simulink model "waypoiont"  (R2026b)
settings: Solver=VariableStepAuto
undefined symbols (not defined in the file): Sim3dSensor
libraries: sim3dcameralib x1, sim3dlib x1, uavsim3dlib x1, uavalgslib x1
settings Model: Creator=Shobhit  LastModifiedBy=Shobhit

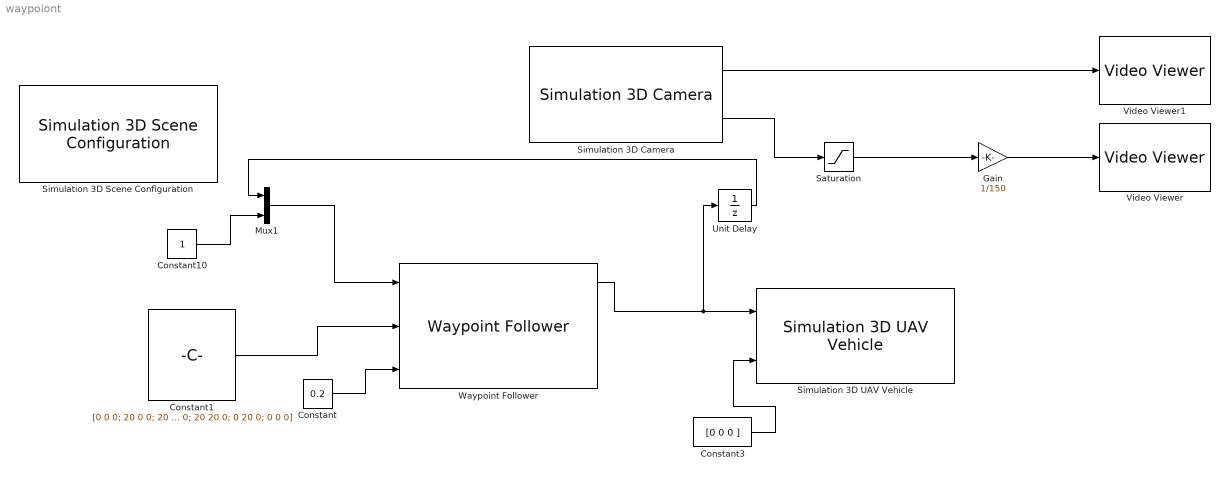
== system waypoiont ==
  Constant : Constant  Value=0.2
  Constant1 : Constant  Value=[0 0 0; 20 0 0; 20 20 0; 0 20 0; 0 0 0; 20 0 0; 20 20 0; 0 20 0; 0 0 0; 20 0 0; 20 20 0; 0 20 0; 0 0 0]
  Constant10 : Constant
  Constant3 : Constant  Value=[0 0 0 ]
  Gain : Gain  Gain=1/150
  Mux1 : Mux  Inputs=2
  Saturation : Saturate  UpperLimit=150  LowerLimit=0
  Simulation 3D Camera : sim3dcameralib/Simulation 3D Camera  Priority=1  sensorTag=Sim3dSensor�  sensorId=4  sensorName=Sim3dSensor�  vehTagList={'Custom ...';'Scene Origin';'SimulinkVehicle3'}  vehTag=SimulinkVehicle3  CoordinateSystem=Default  mountLoc=Origin  offsetFlag=off  tmountOffset=[0, 0, 0]  extTmount=off  rmountOffset=[0, 0, 0]  extRmount=off  FocalLength=[1109, 1109]  OpticalCenter=[640, 360]  ImageSize=[720, 1280]  RadialDistortion=[0, 0]  TangentialDistortion=[0, 0]  SensorSkew=0  VisualizeFieldOfView=off  FieldOfViewRange=61  DepthOutportEnabled=on  SemanticOutportEnabled=off  TransformOutportEnabled=off  SampleTime=-1  mountPoint=[0 0 0]  mountOrientation=[0 0 0]  aMode=5  ID=4
      settings: LibrarySourceBlock=sl3dlib/Simulation 3D/Sensors/Simulation 3D Camera
  Simulation 3D Scene Configuration : sim3dlib/Simulation 3D Scene Configuration  Priority=0  EnableWindow=on  ViewerType=Default Viewer  ProjectFormat=Default Scenes  SceneDesc=US city block  ProjectName=C:\Program Files\MATLAB\R2026b\toolbox\shared\sim3d_projects\automotive_project_windows\UE\WindowsNoEditor\VehicleSimulation.exe  ScenePath=/Game/Maps/USCityBlock  EnableOpenDRIVE=off  vehTagList={'Custom';'Scene Origin';'SimulinkVehicle1';'SimulinkVehicle2';'SimulinkVehicle3'}  vehTag=SimulinkVehicle3  AttachedCameraRelativeTranslation=[0 0 0]  FreeCameraDefaultInitialTranslation=[-6, 0, 2]  AttachedCameraRelativeRotation=[0, -15, 0]  FreeCameraDefaultInitialRotation=[0, -15, 0]  ViewpointName=Custom  FreeCameraInitialTranslation=[0, 0, 0]  FreeCameraInitialRotation=[0, 0, 0]  OpVisEn=off  Ts=1/60  EnableRemoteAccess=off  SimulationMode=CoSimulation  SimulateUsing=Interpreted execution  EnableAnimationRecording=off  OverrideDefaultRecording=off  AnimationRecordingFileName=sim3dAnimation.mat  AnimationRecordingInterval=[0 inf]  EnableWeather=off  SunAzimuth=90  SunAltitude=40.0  EnableGeospatialSun=off  Latitude=0  Longitude=0  Date=2023-01-01  Time=10:30:00  GeoTimeZone=-5.0  SunDaylightSaving=off  wind=1  clouds=10  EnableVolumetricClouds=off  CloudCoverage=0  CloudAltitude=6  fog=0  rain=0  RaindropsEffect=off  SnowDensity=0  EnableGeospatial=off  TilesetSource=Earth terrain  UseTrueOrigin=off  OriginHeight=200  OriginLatitude=40.744652  OriginLongitude=-73.988864  MapStyle=Aerial  AdditionalAssetIDs=[]  UseAdvancedSunSky=off  SolarTime=11  TimeZone=-5  Day=21  Month=9  Year=2022  UseDaylightSavingTime=on  DSTStartDay=10  DSTStartMonth=3  DSTEndDay=3  DSTEndMonth=11  DSTSwitchHour=2  sensorTag=MainCamera3  sensorId=3  sensorName=MainCamera3  mountLoc=Origin  offsetFlag=off  tmountOffset=[0, 0, 0]  rmountOffset=[0, 0, 0]  HorizontalResolution=1280  VerticalResolution=720  HorizontalFOV=60  mountPoint=[0 0 0]  mountOrientation=[0 0 0]  aMode=4  ID=3  GeoTrigger=Inactive  ViewNameList={'Custom'}  ViewTranslationList={'[0 0 0]'}  ViewRotationList={'[0 0 0]'}
      settings: LibrarySourceBlock=uavsim3dlib/Simulation 3D Scene Configuration
  Simulation 3D UAV Vehicle : uavsim3dlib/Simulation 3D UAV Vehicle  Priority=-1  Mesh=Quadrotor  MeshPath=/MathWorksUAVContent/UAVs/HexaRotorUAV/HexaRotor.HexaRotor  Color=Black  ActorName=SimulinkVehicle3  UseGlobalFrame=off  InitialTranslation=[0 0 0]  InitialRotation=[0 0 0]  InitialTranslationGlobal=[0 0 0]  InitialGeoOrigin=[0 0 0]  InitialRotationGlobal=[0 0 0]  SampleTime=-1  ActorType=SimulinkVehicle  ID=3  aMode=4  ActorTag=SimulinkVehicle3
  Unit Delay : UnitDelay  SampleTime=-1
  Video Viewer : VideoViewer  FigPos=[1282 1389 1278 588]
  Video Viewer1 : VideoViewer  FigPos=[5 1399 1350 639]
  Waypoint Follower : uavalgslib/Waypoint Follower  UAVType=multirotor  StartFrom=first  TransitionRadiusSource=internal  TransitionRadius=10  MinLookaheadDistance=0.1  HoverAtLastWaypoint=on  InterpolateYaw=on  YawInput=off  ShowCrossTrackErrorOutput=off  ShowStatusOutput=off  ShowWaypointIndexOutput=off  SimulateUsing=Interpreted execution
  wires:
  Simulation 3D Camera/2 -> Saturation/1
  Saturation/1 -> Gain/1
  Gain/1 -> Video Viewer/1
  Simulation 3D Camera/1 -> Video Viewer1/1
  Constant3/1 -> Simulation 3D UAV Vehicle/2
  Constant10/1 -> Mux1/2
  Unit Delay/1 -> Mux1/1
  Constant/1 -> Waypoint Follower/3
  Constant1/1 -> Waypoint Follower/2
  Mux1/1 -> Waypoint Follower/1
  Waypoint Follower/1 -> Simulation 3D UAV Vehicle/1, Unit Delay/1
